simulink model "VN300_Test"  (R2026b)
settings: Solver=VariableStepAuto
undefined symbols (not defined in the file or in its folder): VN300Config
settings Model: Creator=11and  LastModifiedBy=11and

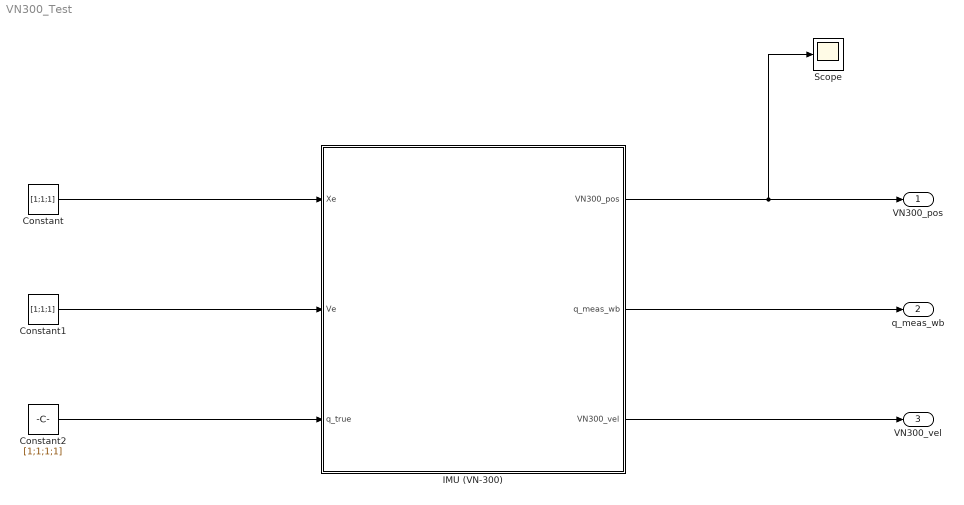
== system VN300_Test ==
  Constant : Constant  Value=[1;1;1]
  Constant1 : Constant  Value=[1;1;1]
  Constant2 : Constant  Value=[1;1;1;1]
  IMU (VN-300) : Subsystem
  Scope : Scope
  VN300_pos : Outport
  q_meas_wb : Outport  Port=2
  VN300_vel : Outport  Port=3
  wires:
  IMU (VN-300)/1(VN300_pos) -> Scope/1, VN300_pos/1
  IMU (VN-300)/3(VN300_vel) -> VN300_vel/1
  IMU (VN-300)/2(q_meas_wb) -> q_meas_wb/1
  Constant/1 -> IMU (VN-300)/1(Xe)
  Constant1/1 -> IMU (VN-300)/2(Ve)
  Constant2/1 -> IMU (VN-300)/3(q_true)

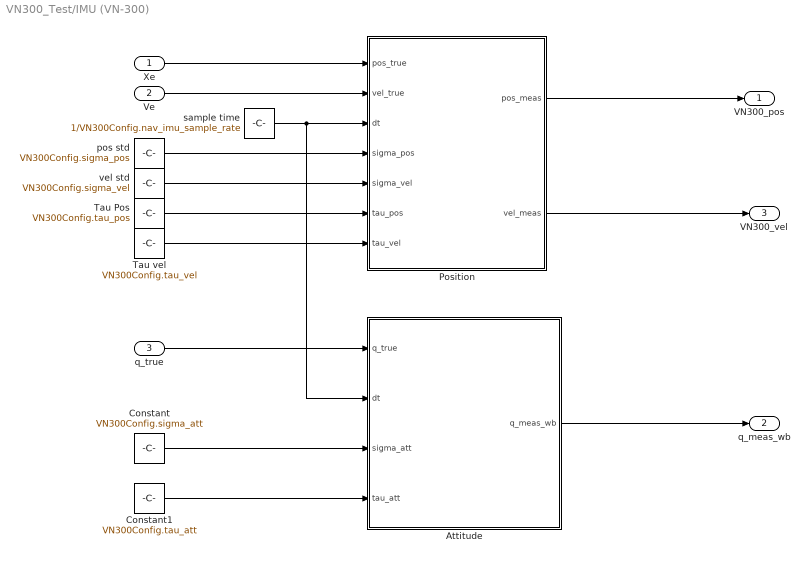
== system VN300_Test/IMU (VN-300) ==
  Xe : Inport
  Ve : Inport  Port=2
  q_true : Inport  Port=3
  Attitude : MATLAB Function  TreatAsAtomicUnit=on  SystemSampleTime=1/VN300Config.nav_imu_sample_rate
  Constant : Constant  Value=VN300Config.sigma_att
  Constant1 : Constant  Value=VN300Config.tau_att
  Position : MATLAB Function  TreatAsAtomicUnit=on  SystemSampleTime=1/VN300Config.nav_imu_sample_rate
  Tau Pos : Constant  Value=VN300Config.tau_pos
  Tau vel : Constant  Value=VN300Config.tau_vel
  pos std : Constant  Value=VN300Config.sigma_pos
  sample time : Constant  Value=1/VN300Config.nav_imu_sample_rate
  vel std : Constant  Value=VN300Config.sigma_vel
  VN300_pos : Outport
  q_meas_wb : Outport  Port=2
  VN300_vel : Outport  Port=3
  wires:
  sample time/1 -> Attitude/2(dt), Position/3(dt)
  Xe/1 -> Position/1(pos_true)
  Ve/1 -> Position/2(vel_true)
  pos std/1 -> Position/4(sigma_pos)
  vel std/1 -> Position/5(sigma_vel)
  Tau Pos/1 -> Position/6(tau_pos)
  Tau vel/1 -> Position/7(tau_vel)
  q_true/1 -> Attitude/1(q_true)
  Attitude/1(q_meas_wb) -> q_meas_wb/1
  Constant/1 -> Attitude/3(sigma_att)
  Constant1/1 -> Attitude/4(tau_att)
  Position/1(pos_meas) -> VN300_pos/1
  Position/2(vel_meas) -> VN300_vel/1

== matlab function VN300_Test/IMU (VN-300)/Position ==
  data: pos_meas output; vel_meas output; pos_true input; vel_true input; dt input; sigma_pos input; sigma_vel input; tau_pos input; tau_vel input
function [pos_meas, vel_meas]= fcn(pos_true, vel_true, dt, sigma_pos, sigma_vel, tau_pos, tau_vel)
% pos = Inertial position ([m,m,m])
% vel = Inertial velocity ([m/s,m/s,m/s])
% dt = VN300 sample time (s)
% sigma_pos = steady-state standard deviation of position (RMS)
% sigma_vel = steady-state standard deviation of velocity (m/s)
% tau_pos = how long error persists (s)
% tau_vel = how long error persists (s)

persistent pos_error vel_error

if isempty(pos_error)
    pos_error = zeros(3,1);
    vel_error = zeros(3,1);
end

%% Time-Correlated Error
% GNSS measurements are time-correlated so errors can arise dependent on sample time
% This model is the first-order Gauss-Markov process
a_pos = exp(-dt/tau_pos);
a_vel = exp(-dt/tau_vel);

%% Total Error
pos_error = a_pos.*pos_error + sigma_pos.*sqrt(1-a_pos.^2).*randn(3,1);
vel_error = a_vel.*vel_error + sigma_vel.*sqrt(1-a_vel.^2).*randn(3,1);

pos_meas = pos_true + pos_error;
vel_meas = vel_true + vel_error;

== matlab function VN300_Test/IMU (VN-300)/Attitude ==
  data: q_true input; q_meas_wb output; dt input; sigma_att input; tau_att input
function q_meas_wb = fcn(q_true, dt, sigma_att, tau_att)
% sigma_att = standard dev of [roll RMS, pitch RMS, heading RMS]
% tau_att = correlation time for attitude (s)

persistent att_error

if isempty(att_error)
    att_error = zeros(3,1);
end

%% Time Correlation 
% Like the position block, we'll use Guass-Markov Process

a = exp(-dt/tau_att);

att_error = a*att_error + sigma_att*sqrt(1-a^2).*randn(3,1);% [rads, rads, rads]

%% Quaternion error
q_error = [1;0.5*att_error]; % small angle approximation
q_error = q_error/norm(q_error); 

q_meas_wb = quatmultiply(q_true',q_error');
q_meas_wb = q_meas_wb/norm(q_meas_wb); % measured quaternion (earth to body)
